simulink model "eml_hdl_design_patterns"  (R2026a)
settings: Solver=FixedStepDiscrete  StopTime=10
InitFcn:
  | errMsg  = ['\n\nThis model is only for demonstration purposes.\n\nPlease do not Simulate or code generate directly from this model. \n\nBefore generating code from this model please do copy the relevant blocks of interest from this model to a new model, place them in a subsystem, build a valid test bench around them.\n\nPlease refer to the example model ''eml_hdl_incrementer'' or HDLCoder documentation'];
  | error(sprintf(errMsg));
undefined symbols (not defined in the file or in its folder): C, gain_val, init_val, lower_limit, maxWordLength, thresh, upper_limit
libraries: simulink x2
(part 3 of 5)

== matlab function eml_hdl_design_patterns/CPU Parts/CPU Controller ==
  settings: sampleTime=1
  settings: fimath=|
      | fimath(...
      | 'RoundMode', 'floor',...
      | 'OverflowMode', 'wrap',...
      | 'ProductMode', 'FullPrecision', 'ProductWordLength', 32,...
      | 'SumMode', 'FullPrecision', 'SumWordLength', 32,...
      | 'CastBeforeSum', true)
  data: data_in input uint8; in_flags input fixdt(0,4,0); master_rst input boolean; shifter_sel output; out_flags output; ALU_func output; print_data output; DM_addr output; DM_r_w output; AC_func output; AC_data output; IR_func output; PC_func output; addr_inc output; IM_read output; hlt output; IR_in input fixdt(0,12,0)
function [shifter_sel, out_flags, ALU_func, ...
    print_data, DM_addr, DM_r_w, AC_func, AC_data, IR_func, ...
    PC_func, addr_inc, IM_read, hlt] = Controller(data_in, in_flags, master_rst, IR_in)
% CPU Controller
%
% The CPU Instruction Set:
% ------------------------
% 
% LDA <loc>: AC = content(<loc>)
% LDAI <loc>: AC = content(content(<loc>))
% AND <loc>: AC = AC & content(<loc>)
% ANDI <loc>: AC = AC & content(content(<loc>))
% ADD <loc>: AC = AC + content(<loc>) + C(flag) 
% ADDI <loc>: AC = AC + content(content(<loc>)) + C(flag)
% SUB <loc>: AC = AC - content(<loc>) - C(flag) 
% SUBI <loc>: AC = AC - content(content(<loc>)) - C(flag)
% JMP <loc>: Jump to <PC + <loc>>
% LI <const>: AC = <const>
% STA <loc>: content(<loc>) = AC
% STAI <loc>: content(content(<loc>)) = AC
% BRA_C <loc>: Jump to <PC + <loc>> if (C(flag) == 1)
% BRA_N <loc>: Jump to <PC + <loc>> if (N(flag) == 1)
% BRA_V <loc>: Jump to <PC + <loc>> if (V(flag) == 1)
% BRA_Z <loc>: Jump to <PC + <loc>> if (Z(flag) == 1)
% NOP: Do nothing
% CLA: AC = 0
% CMA: Complement AC
% CMC: Complement C(flag)
% ASL: AC = AC << 1
% ASR: AC = AC >> 1
% PRINT: Display value from the memory-mapped location 254
% CLC: C(flag) = 0
%
% 12-bit Instruction Encoding:
% ---------------------------
%
% 	LDA:   000 0 <8-bit loc>
% 	LDAI:  000 1 <8-bit loc>
% 	AND:   001 0 <8-bit loc>
% 	ANDI:  001 1 <8-bit loc>
% 	ADD:   010 0 <8-bit loc>
% 	ADDI:  010 1 <8-bit loc>
% 	SUB:   011 0 <8-bit loc>
% 	SUBI:  011 1 <8-bit loc>
% 	JMP:   1000 <8-bit loc>
% 	LI:    1001 <8-bit const>
% 	STA:   101 0 <8-bit loc>
% 	STAI:  101 1 <8-bit loc>
% 	BRA_C: 1100 <8-bit loc>
% 	BRA_N: 1101 <8-bit loc>
% 	BRA_C: 1110 <8-bit loc>
% 	BRA_C: 1111 <8-bit loc>
% 	HLT:   111 0 0100 0 000 
% 	CLA:   111 0 0100 1 000
% 	CMA:   111 0 0101 0 000
% 	CMC:   111 0 0101 1 000
% 	ASL:   111 0 0110 0 000
% 	ASR:   111 0 0110 1 000
% 	PRINT: 111 0 0111 0 000
% 	CLC:   111 0 0111 1 000  

% HDL specific fimath
hdl_fm = fimath(...
'RoundMode', 'floor',...
'OverflowMode', 'wrap',...
'ProductMode', 'FullPrecision', 'ProductWordLength', 32,...
'SumMode', 'FullPrecision', 'SumWordLength', 32,...
'CastBeforeSum', true);


persistent CPU_state;
if(isempty(CPU_state))
    CPU_state = uint8(0);
end

if(master_rst)
    CPU_state = uint8(0);
end

shifter_sel = fi(0, 0, 2, 0, hdl_fm);
ALU_func = fi(0, 0, 3, 0, hdl_fm);
out_flags = in_flags;
AC_func = fi(4, 0, 3, 0, hdl_fm);  % NOP
AC_data = fi(0, 1, 8, 0, hdl_fm);
IR_func = fi(3, 0, 2, 0, hdl_fm);  % NOP
PC_func = fi(3, 0, 2, 0, hdl_fm);  % NOP
IM_read = fi(0, 0, 1, 0, hdl_fm);
DM_addr = uint8(0);
DM_r_w = fi(0, 0, 2, 0, hdl_fm);
addr_inc = fi(0, 1, 8, 0, hdl_fm);
print_data = false;
hlt = uint8(0);

% Instruction: <12..1>
% major_opcode: <12..10>
% indirect_addressing: <9>
% minor_opcode: <9..4>
% address bits: <8..1>

persistent major_opcode; 
persistent minor_opcode; 
persistent address_data;

if(isempty(major_opcode))
    major_opcode = fi(0, 0, 8, 0, hdl_fm);
    minor_opcode = fi(0, 0, 8, 0, hdl_fm);
    address_data = fi(0, 0, 8, 0, hdl_fm);
end

switch(CPU_state)
    %%%%%%%%%%%%%%%%%%%%%%%%%%%%%%%%%%%%%%
    %  RESETTING OUTPUTS
    %%%%%%%%%%%%%%%%%%%%%%%%%%%%%%%%%%%%%%
    case 0
        PC_func = fi(0, 0, 2, 0, hdl_fm);   
        AC_func = fi(0, 0, 3, 0, hdl_fm);   
        IR_func = fi(0, 0, 2, 0, hdl_fm);   
        CPU_state = uint8(1);
        
    %%%%%%%%%%%%%%%%%%%%%%%%%%%%%%%%%%%%%%
    %  FETCH
    %%%%%%%%%%%%%%%%%%%%%%%%%%%%%%%%%%%%%%
    case 1 
        % Read from IM
        IM_read = fi(1, 0, 1, 0, hdl_fm);  
        % Increment PC
        PC_func = fi(2, 0, 2, 0, hdl_fm);  
        % store into IR
        IR_func = fi(1, 0, 2, 0, hdl_fm);  
        CPU_state = uint8(2);
        
    case 2 
        % Read from IR
        IR_func = fi(2, 0, 2, 0, hdl_fm);  
        % Accommodating for the 'unit delay' from IR_out to IR_in
        CPU_state = uint8(3);  
        
    case 3
        % IR_in <12..10>
        major_opcode = fi(bitsrl(IR_in, 9), 0, 8, 0, hdl_fm);
        mask = fi(63, 0, 12, 0, hdl_fm);
        % IR_in <9..4>
        minor_opcode = fi(bitand(bitsrl(IR_in, 3), mask), 0, 8, 0, hdl_fm);
        mask = fi(255, 0, 12, 0, hdl_fm);
        % IR_in <8..1>
        address_data = fi(bitand(IR_in, mask), 0, 8, 0, hdl_fm);
        
        % Go to the decode stage
        CPU_state = uint8(4);  
        
    %%%%%%%%%%%%%%%%%%%%%%%%%%%%%%%%%%%%%%
    %  DECODE AND EXECUTE
    %%%%%%%%%%%%%%%%%%%%%%%%%%%%%%%%%%%%%%
    case 4  
        switch(uint8(major_opcode))
            case 0  
                % LDA
                % minor_opcode contains the address (assuming direct addressing)
                DM_addr = uint8(address_data); 
                % Read the data memory
                DM_r_w = fi(2, 0, 2, 0, hdl_fm); 
                % Simply pass the value read from memory
                ALU_func = fi(6, 0, 3, 0, hdl_fm); 
                shifter_sel = fi(3, 0, 2, 0, hdl_fm); 
                
                indirect_bit = bitget(minor_opcode, 6);
                
                if(logical(indirect_bit))
                    % indirect addressing
                    CPU_state = uint8(7);
                else
                    CPU_state = uint8(6);
                end
                
            case 1  
                % AND           
                DM_addr = uint8(address_data);
                % Reading the data memory for address or data
                DM_r_w = fi(2, 0, 2, 0, hdl_fm);
                indirect_bit = bitget(minor_opcode, 6);
                if(logical(indirect_bit))
                    % indirect addressing
                    CPU_state = uint8(8);
                else
                    % Performing AND
                    ALU_func = fi(1, 0, 3, 0, hdl_fm);
                    shifter_sel = fi(3, 0, 2, 0, hdl_fm);
                    CPU_state = uint8(6);
                end
                
            case 2  
                % ADD
                DM_addr = uint8(address_data);
                % Reading the data memory for address or data
                DM_r_w = fi(2, 0, 2, 0, hdl_fm);
                indirect_bit = bitget(minor_opcode, 6);
                if(logical(indirect_bit))
                    % indirect addressing
                    CPU_state = uint8(9);
                else
                    % Performing ADD
                    ALU_func = fi(2, 0, 3, 0, hdl_fm); 
                    shifter_sel = fi(3, 0, 2, 0, hdl_fm);
                    CPU_state = uint8(6);
                end 
                
            case 3  
                % SUB
                DM_addr = uint8(address_data);
                % Reading the data memory for address or data
                DM_r_w = fi(2, 0, 2, 0, hdl_fm);
                indirect_bit = bitget(minor_opcode, 6);
                if(logical(indirect_bit))
                    % indirect addressing
                    CPU_state = uint8(10);
                else
                    % Performing SUB
                    ALU_func = fi(3, 0, 3, 0, hdl_fm); 
                    shifter_sel = fi(3, 0, 2, 0, hdl_fm);
                    CPU_state = uint8(6);
                end 

            case 4  
                minor_opcode_bit6 = bitget(minor_opcode, 6);
                switch(uint8(minor_opcode_bit6))
                    case 0 
                        % JMP
                        temp_address_data = fi(address_data, 1, 7, 0, hdl_fm);
                        addr_inc = fi(temp_address_data-1, 1, 8, 0, hdl_fm);
                        PC_func = fi(1, 0, 2, 0, hdl_fm); 
                        
                    case 1
                        % LI
                        AC_data = fi(address_data, 1, 8, 0, hdl_fm);
                        AC_func = fi(1, 0, 3, 0, hdl_fm);
                end
                % Go back to the fetch stage again
                CPU_state = uint8(1);  
                
            case 5  
                % STA
                % minor_opcode contains the address (assuming direct addressing)
                DM_addr = uint8(address_data); 
                indirect_bit = bitget(minor_opcode, 6);
                if(logical(indirect_bit))
                    % indirect addressing
                    % Read the address from the data memory
                    DM_r_w = fi(2, 0, 2, 0, hdl_fm); 
                    CPU_state = uint8(11);
                else
                    % Write into the data memory
                    DM_r_w = fi(1, 0, 2, 0, hdl_fm);
                    % Go back to the fetch stage again
                    CPU_state = uint8(1);
                end
                
            case 6
                minor_opcode_bit6 = bitget(minor_opcode, 6);
                switch(uint8(minor_opcode_bit6))
                    % special branches:
                    case 0 
                        % BRA_C
                        c = bitget(in_flags, 4);
                        if(logical(c))
                            temp_address_data = fi(address_data, 1, 7, 0, hdl_fm);
                            addr_inc = fi(temp_address_data-1, 1, 8, 0, hdl_fm);
                            PC_func = fi(1, 0, 2, 0, hdl_fm);
                        end
                        
                    case 1
                        % BRA_N
                        n = bitget(in_flags, 3);
                        if(logical(n))
                            temp_address_data = fi(address_data, 1, 7, 0, hdl_fm);
                            addr_inc = fi(temp_address_data-1, 1, 8, 0, hdl_fm);
                            PC_func = fi(1, 0, 2, 0, hdl_fm);
                        end
                end
                % Go back to the fetch stage again
                CPU_state = uint8(1);
                
            case 7  
                 % by default, go back to the fetch stage again
                CPU_state = uint8(1);
                minor_opcode_bit4 = bitget(minor_opcode, 4);
                if(logical(minor_opcode_bit4) == 0)
                    % Further cases of special branches:
                    minor_opcode_bit6 = bitget(minor_opcode, 6);
                    switch(uint8(minor_opcode_bit6))
                        case 0 
                            % BRA_V
                            v = bitget(in_flags, 2);
                            if(logical(v))
                                temp_address_data = fi(address_data, 1, 7, 0, hdl_fm);
                                addr_inc = fi(temp_address_data-1, 1, 8, 0, hdl_fm);
                                PC_func = fi(1, 0, 2, 0, hdl_fm);
                            end
                         
                        case 1 
                            % BRA_Z
                            z = bitget(in_flags, 1);
                            if(logical(z))
                                temp_address_data = fi(address_data, 1, 7, 0, hdl_fm);
                                addr_inc = fi(temp_address_data-1, 1, 8, 0, hdl_fm);
                                PC_func = fi(1, 0, 2, 0, hdl_fm);
                            end
                    end
                end
                % Instructions having no operands
                switch(uint8(minor_opcode))
                    case 8
                        % HLT
                        % Stop the simulation
                        hlt = uint8(1);
                        CPU_state = uint8(1);
                    case 9 
                        % CLA
                        AC_func = fi(0, 0, 3, 0, hdl_fm);
                        
                    case 10 
                        % CMA
                        ALU_func = fi(4, 0, 3, 0, hdl_fm); 
                        shifter_sel = fi(3, 0, 2, 0, hdl_fm);
                        CPU_state = uint8(6);
                        
                    case 11 
                        % CMC
                        ALU_func = fi(5, 0, 3, 0, hdl_fm); 
                        shifter_sel = fi(3, 0, 2, 0, hdl_fm);
                        
                    case 12 
                        % ASL
                        shifter_sel = fi(1, 0, 2, 0, hdl_fm);
                        CPU_state = uint8(6);
                        
                    case 13 
                        % ASR
                        shifter_sel = fi(2, 0, 2, 0, hdl_fm);
                        CPU_state = uint8(6);
                        
                    case 14 
                        % PRINT
                        print_data = true;
                        
                    case 15 
                        % CLC
                        ALU_func = fi(7, 0, 3, 0, hdl_fm); 
                        shifter_sel = fi(3, 0, 2, 0, hdl_fm);
                        
                    otherwise
                        % by default, go back to the fetch stage again
                        CPU_state = uint8(1);
  
                % Minor Opcode cases end here        
                end
        % Major Opcode cases end here
        end
    
    % introducing delay
    case 6
        % accounting for the delay from shift_out to AC_in2
        AC_func = fi(2, 0, 3, 0, hdl_fm);
        % Go back to the fetch stage again
        CPU_state = uint8(1);  
        
    % Operations with indirect addressing
    case 7
        % LDA Indirect
        % data_in is the address read from the data memory
        DM_addr = uint8(data_in); 
        % Read the data memory
        DM_r_w = fi(2, 0, 2, 0, hdl_fm); 
        % Simply pass the value read from memory
        ALU_func = fi(6, 0, 3, 0, hdl_fm); 
        shifter_sel = fi(3, 0, 2, 0, hdl_fm); 
        % accounting for the algebraic loop delay        
        CPU_state = uint8(6);
        
    case 8
        % AND Indirect
        % data_in is the address read from the data memory
        DM_addr = uint8(data_in);
        % Read the data memory
        DM_r_w = fi(2, 0, 2, 0, hdl_fm);
        % Performing AND
        ALU_func = fi(1, 0, 3, 0, hdl_fm);
        shifter_sel = fi(3, 0, 2, 0, hdl_fm);
        % accounting for the algebraic loop delay
        CPU_state = uint8(6);
    
    case 9
        % ADD Indirect
        % data_in is the address read from the data memory
        DM_addr = uint8(data_in);
        % Read the data memory
        DM_r_w = fi(2, 0, 2, 0, hdl_fm);
        % Performing ADD
        ALU_func = fi(2, 0, 3, 0, hdl_fm); 
        shifter_sel = fi(3, 0, 2, 0, hdl_fm);
        % accounting for the algebraic loop delay
        CPU_state = uint8(6);
        
    case 10
        % SUB Indirect
        % data_in is the address read from the data memory
        DM_addr = uint8(data_in);
        % Read the data memory
        DM_r_w = fi(2, 0, 2, 0, hdl_fm);
        % Performing SUB
        ALU_func = fi(3, 0, 3, 0, hdl_fm); 
        shifter_sel = fi(3, 0, 2, 0, hdl_fm);
        % accounting for the algebraic loop delay
        CPU_state = uint8(6);
        
    case 11
        % STA Indirect
        % data_in is the address read from the data memory
        DM_addr = uint8(data_in);
        % Write the data memory
        DM_r_w = fi(1, 0, 2, 0, hdl_fm);
        CPU_state = uint8(1);
        
    otherwise
        % by default, go back to the fetch stage again
        CPU_state = uint8(1);
                
% switch(CPU_state) end here
end

== matlab function eml_hdl_design_patterns/Misc/const_typing/untyped ==
  settings: fimath=|
      | fimath(...
      | 'RoundMode', 'floor',...
      | 'OverflowMode', 'wrap',...
      | 'ProductMode', 'FullPrecision', 'ProductWordLength', 32,...
      | 'SumMode', 'FullPrecision', 'SumWordLength', 32,...
      | 'CastBeforeSum', true)
  data: u input fixdt(1,14,3); y output
function y = fcn(u)

% based on the internal rule that 
% computes output type gives 
% non-optimial result type (sfix24_En12)

y = u + 1;

== matlab function eml_hdl_design_patterns/Misc/const_typing/typed ==
  settings: fimath=|
      | fimath(...
      | 'RoundMode', 'floor',...
      | 'OverflowMode', 'wrap',...
      | 'ProductMode', 'FullPrecision', 'ProductWordLength', 32,...
      | 'SumMode', 'FullPrecision', 'SumWordLength', 32,...
      | 'CastBeforeSum', true)
  data: u input fixdt(1,14,3); y1 output; y2 output
function [y1, y2] = fcn(u)

% choose minimal required for const 1
y1 = u + fi(1, 0, 1, 0, fimath(u));

% choose same type as var u
y2 = u + fi(1, numerictype(u), fimath(u));

% 
% you get optimal result types (sfix15_En3)
% when you explicitly choose constant types
%
% IMP: Also do not forget to choose 'FullPrecision' 
% on 'Product' and 'SumModes' in the fimath settings
% of this block

== matlab function eml_hdl_design_patterns/Comparators/eml_tree_min ==
  settings: fimath=|
      | fimath(...
      | 'RoundMode', 'floor',...
      | 'OverflowMode', 'wrap',...
      | 'ProductMode', 'FullPrecision', 'ProductWordLength', 32,...
      | 'SumMode', 'FullPrecision', 'SumWordLength', 32,...
      | 'CastBeforeSum', true)
  data: invec input fixdt(1,12,6) size=64; minval output; idx output uint32
%--------------------------------------------------------------------------
% Tree implementation min function for vector input of length 64
%--------------------------------------------------------------------------
function [minval, idx] = fcn(invec)

% initialize outputs
minval = gethdlfi(0, 1, 12, 6);
idx = uint32(0);

% first level of comparison
inidx = uint32(1:64);
[lvlonemin, lvloneidx] = vector_min(invec, inidx);

% second level of comparison
[lvltwomin, lvltwoidx] = vector_min(lvlonemin, lvloneidx);

% third level of comparison
[lvlthreemin, lvlthreeidx] = vector_min(lvltwomin, lvltwoidx);

% fourth level of comparison
[lvlfourmin, lvlfouridx] = vector_min(lvlthreemin, lvlthreeidx);

% fifth level of comparison
[lvlfivemin, lvlfiveidx] = vector_min(lvlfourmin, lvlfouridx);

% final comparison
[minval, idx] = vector_min(lvlfivemin, lvlfiveidx);


end

% Minimum subfuction for tree implementation
function [minvec, idxvec] = vector_min(invec, inidx)
    
lengthminvec = uint8(length(invec)/2);
minvec = gethdlfi(zeros(lengthminvec, 1), 1, 12, 6);
idxvec = uint32(zeros(lengthminvec, 1));

for i=1:lengthminvec
    % get two consecutive values
    idx2 = int8(i)+int8(i); %i*2
    idx1 = int8(idx2) - int8(1); %i*2-1
    % get elements
    val1 = invec(idx1);
    val2 = invec(idx2);
    % compare them and select minimum
    if val1 <= val2
        minvec(i) = val1;
        idxvec(i) = inidx(idx1);
    else
        minvec(i) = val2;
        idxvec(i) = inidx(idx2);
    end
end

end


function myfi = gethdlfi(input, issigned, wlen, flen)

fm = fimath(...
    'RoundMode', 'floor',...
    'OverflowMode', 'wrap',...
    'ProductMode', 'FullPrecision', 'ProductWordLength', 32,...
    'SumMode', 'FullPrecision', 'SumWordLength', 32,...
    'CastBeforeSum', true);

myfi = fi(input, issigned, wlen, flen, 'fimath', fm);

end

== matlab function eml_hdl_design_patterns/Complex/Real Imag To Complex ==
  settings: fimath=|
      | fimath(...
      | 'RoundMode', 'floor',...
      | 'OverflowMode', 'wrap',...
      | 'ProductMode', 'FullPrecision', 'ProductWordLength', 32,...
      | 'SumMode', 'FullPrecision', 'SumWordLength', 32,...
      | 'CastBeforeSum', true)
  data: re input; c output; im input
function c = fcn(re, im)
% Convert real and/or imaginary inputs to complex signal
%
% This Real-Imag to Complex function converts real and/or imaginary inputs
% to a complex-valued output signal.
%
% The inputs can both be arrays (vectors) of equal dimensions, 
% or one input can be an array and the other a scalar. If the function 
% has an array input, the output is a complex array of the 
% same dimensions. 
%
% The elements of the real input are mapped to the real parts of the 
% corresponding complex output elements. The imaginary input is similarly 
% mapped to the imaginary parts of the complex output signals. 
% If one input is a scalar, it is mapped to the corresponding component 
% (real or imaginary) of all the complex output signals. 
%
% The input signals and real or imaginary output parameter can be of any
% data type supported by Simulink, except Boolean. The Real-Imag
% to Complex block supports fixed-point data types. The output is of 
% the same type as the input or parameter that determines the output.

c = complex(re, im);

== matlab function eml_hdl_design_patterns/Misc/eml_expr ==
  settings: fimath=|
      | fimath(...
      | 'RoundMode', 'ceil',...
      | 'OverflowMode', 'saturate',...
      | 'ProductMode', 'FullPrecision', 'ProductWordLength', 32,...
      | 'SumMode', 'FullPrecision', 'SumWordLength', 32,...
      | 'CastBeforeSum', true)
  data: a input fixdt(1,5,2); y output fixdt(1,7,4); b input fixdt(1,5,3)
function y = fcn(a,b)

%------------------------ BLOCK COMMENTS BEGIN ------------------------
%
% The following fixpt expression 
%
%       y = fi((a*b) - (a+b), 1, 7, 4);
%
% with operand and output types 
%
%     a (sfix5_En2), b (sfix5_En3),  y (sfix7_En4) 
%
% and with default fixpt settings on the eML block (ceil,saturate)
%
%  fimath(...
%   'RoundMode', 'ceil',...
%   'OverflowMode', 'saturate',...
%   'ProductMode', 'FullPrecision', 'ProductWordLength', 32,...
%   'SumMode', 'FullPrecision', 'SumWordLength', 32,...
%   'CastBeforeSum', true)
%
% should generate the HDL code based on following intermediate result types
%
%      tmul = a*b (sfix10_En5)
% 
%      t2 = (sfix7_En3) a
%      t3 = (sfix7_En3) b
% 
%      tadd = t2 + t3;
% 
%      t4 = (sfix11_En5) tmul;
%      t5 = (sfix11_En5) tadd;
% 
%      tsub = t4 - t5
% 
%      y = (sfix7_En4) tsub;
% 
%  
%------------------------ BLOCK COMMENTS END ------------------------


% fixpt arithmetic expression
expr = (a*b) - (a+b);

% cast the result to correct output type
y = fi(expr, 1, 7, 4);

== matlab function eml_hdl_design_patterns/CPU Parts/Data Memory (256-Bytes) ==
  settings: sampleTime=1
  settings: fimath=|
      | fimath(...
      | 'RoundMode', 'floor',...
      | 'OverflowMode', 'wrap',...
      | 'ProductMode', 'FullPrecision', 'ProductWordLength', 32,...
      | 'SumMode', 'FullPrecision', 'SumWordLength', 32,...
      | 'CastBeforeSum', true)
  data: indirect input boolean; print_data input boolean; ext_out output; addr input uint8; read_write input fixdt(0,2,0); data_out output fixdt(1,8,0); data_in input fixdt(1,8,0)
function [ext_out, data_out] = fcn(indirect, print_data, addr, read_write, data_in)
% An 8-bit byte-addressable Data Memory
% read_write == 1 => write into DM
% read_write == 2 => read from DM
% print_data == 1 => print data out from memory location 32
% indirect == 1 => Indirect addressing, otherwise direct

% HDL specific fimath
hdl_fm = fimath(...
'RoundMode', 'floor',...
'OverflowMode', 'wrap',...
'ProductMode', 'FullPrecision', 'ProductWordLength', 32,...
'SumMode', 'FullPrecision', 'SumWordLength', 32,...
'CastBeforeSum', true);


persistent data;
if(isempty(data))
    data = fi(zeros(1, 256), 1, 8, 0, hdl_fm);
end

% Data in memory
% data(1) = fi(5, 1, 8, 0, hdl_fm);
% data(2) = fi(6, 1, 8, 0, hdl_fm);

% Get the data for indirect referencing
mem_data = data(addr+1);

% Storing data in memory
if(read_write == 1)
    if(indirect)
        % indirect addressing
        new_addr = uint8(mem_data);
        data(new_addr+1) = data_in;
    else
        % direct addressing
        data(addr+1) = data_in;
    end
end


data_out = fi(0, 1, 8, 0, hdl_fm); 

% Loading from memory
if(read_write == 2)
    if(indirect)
        % indirect addressing
        new_addr = uint8(mem_data);
        data_out = data(new_addr + 1);
    else
        % direct addressing
        data_out = mem_data;
    end
end


ext_out = fi(0, 1, 8, 0, hdl_fm);  

% Printing data out from memory location 256 (memory mapped)
if(print_data)
    ext_out = data(255);
end

== matlab function eml_hdl_design_patterns/Adders/ripple_adder ==
  settings: fimath=|
      | fimath(...
      | 'RoundMode', 'floor',...
      | 'OverflowMode', 'wrap',...
      | 'ProductMode', 'FullPrecision', 'ProductWordLength', 32,...
      | 'SumMode', 'FullPrecision', 'SumWordLength', 32,...
      | 'CastBeforeSum', true)
  data: a input fixdt(0,4,0); s output; b input fixdt(0,4,0); carry output
function [s,carry] = fcn(a,b)

% assuming input is of type ufix4

% An and Bn are typically 1-bit
%(but conceptually can be n-bit numbers)

% each adder adds a delay!

nt = numerictype(0, 1, 0);
fm = fimath(a);

a0 = bitsliceget(a, 1, 1);
a1 = bitsliceget(a, 2, 2);
a2 = bitsliceget(a, 3, 3);
a3 = bitsliceget(a, 4, 4);

b0 = bitsliceget(b, 1, 1);
b1 = bitsliceget(b, 2, 2);
b2 = bitsliceget(b, 3, 3);
b3 = bitsliceget(b, 4, 4);

c_in = fi(0, nt, fm);

% add lsb bits
[s0, c0] = bit_adder(a0, b0, c_in);
% add bits at position '1'
[s1, c1] = bit_adder(a1, b1, c0);
% add bits at position '2'
[s2, c2] = bit_adder(a2, b2, c1);
% add msb bits
[s3, c3] = bit_adder(a3, b3, c2);

% form the final sum
s = bitconcat(bitconcat(bitconcat(s3, s2), s1), s0);

% final carry;
carry = c3;

function [s, c] = bit_adder(abit, bbit, cbit)

r = abit + bbit + cbit;

nt = numerictype(abit);
fm = fimath(abit);

s = fi(bitsliceget(r, 1, 1), nt, fm);
c = fi(bitsliceget(r, 2, 2), nt, fm);

== matlab function eml_hdl_design_patterns/CPU Parts/Arithmetic Logical Unit (8-bit) ==
  settings: sampleTime=1
  settings: fimath=|
      | fimath(...
      | 'RoundMode', 'floor',...
      | 'OverflowMode', 'wrap',...
      | 'ProductMode', 'FullPrecision', 'ProductWordLength', 32,...
      | 'SumMode', 'FullPrecision', 'SumWordLength', 32,...
      | 'CastBeforeSum', true)
  data: in_flags input fixdt(0,4,0); func input fixdt(0,3,0); alu_in input fixdt(1,8,0); AC input fixdt(1,8,0); alu_out output fixdt(1,8,0); out_flags output
function [alu_out, out_flags] = ALU(in_flags, func, alu_in, AC)
% This 8-bit ALU supports the following operations:
% AND (Logical AND), ADD, SUB, CMA (Complement AC), CMC (Complement Carry) and CLC (Clear Carry)
% and appropriately sets a 4-bit flag register, which has the following format:
% [C N V Z]

% HDL specific fimath
hdl_fm = fimath(...
'RoundMode', 'floor',...
'OverflowMode', 'wrap',...
'ProductMode', 'FullPrecision', 'ProductWordLength', 32,...
'SumMode', 'FullPrecision', 'SumWordLength', 32,...
'CastBeforeSum', true);

% Get the carry in
carry = bitsliceget(in_flags, 4, 4); 

% Get the overflow in
overflow = bitsliceget(in_flags, 2, 2);

% Simply pass the AC, when there is no designated func
alu_out = fi(AC, 1, 8, 0, hdl_fm);

% 3-bit encoding of ALU ops, which can potentially support upto 8 operations
% Most of the encodings are unused to comply to Parwan supported ops
switch(uint8(func))
    case 0 % NOP
        % simply pass the AC
    case 1 % AND
        % Bitwise AND
        alu_out = bitand(alu_in, AC);
    case 2 % ADD
        % Add with carry and overflow appropriately set
        [alu_out, carry, overflow] = sum_w_carry(AC, alu_in, carry);
    case 3 % SUB
        % Subtract with borrow (set to carry) and overflow appropriately set
        [alu_out, carry, overflow] = sub_w_borrow(AC, alu_in, carry);
    case 4 % CMA
        % Complement AC
        alu_out = fi(bitcmp(AC), 1, 8, 0, hdl_fm);
    case 5 % CMC
        % Complement Carry
        carry = bitcmp(carry);
    case 6 % Get alu_in out
        % Pass the input
        alu_out = fi(alu_in, 1, 8, 0, hdl_fm);
    case 7 % CLC
        % Clear Carry
        carry = fi(0, 0, 1, 0, hdl_fm); 
end

% Negativity  (N)
sign_bit = getmsb(alu_out); 

% Is Zero? (Z)
is_zero = uint8(~all(alu_out));
zero_ufix1 = fi(is_zero, 0, 1, 0, hdl_fm);

% Set the output flag register [C N V Z]
out_flags = bitconcat(bitconcat(bitconcat(carry, sign_bit), overflow), zero_ufix1);

%%%%%%%%%%%%%%%%%%%%%%%%%%%%%%%%%%%%%%%%%%%%%%%%%%%%%%%%%%%%%%%%


%% Full Subtracter with flag register appropriately set 
% diff = u1 - u2 - b_in = u1 + bitcmp(u2) + bitcmp(b_in)
% appropriately set the borrow and the overflow
function [diff, carry, overflow] = sub_w_borrow(u1, u2, b_in)

[diff, carry, overflow] = sum_w_carry(u1, bitcmp(u2), bitcmp(b_in));
%%%%%%%%%%%%%%%%%%%%%%%%%%%%%%%%%%%%%%%%%%%%%%%%%%%%%%%%%%%%%%%%


%% Full Adder with flag register appropriately set
% sum = u1 + u2 + c_in
% appropriately set the carry and the overflow
function [sum, carry, overflow] = sum_w_carry(u1, u2, c_in)

hdl_fm = fimath(...
'RoundMode', 'floor',...
'OverflowMode', 'wrap',...
'ProductMode', 'FullPrecision', 'ProductWordLength', 32,...
'SumMode', 'FullPrecision', 'SumWordLength', 32,...
'CastBeforeSum', true);

% zero-extend u1 by 1 bit for carry detection
temp_u1 = fi(bitconcat(fi(0, 0, 1, 0, hdl_fm), u1), 1, 9, 0, hdl_fm);

% zero-extend u2 by 1 bit for carry detection
temp_u2 = fi(bitconcat(fi(0, 0, 1, 0, hdl_fm), u2), 1, 9, 0, hdl_fm);

% Sum is stored in 9 bits with the msb indicating carry
temp_sum = fi(temp_u1 + temp_u2 + c_in, 1, 9, 0, hdl_fm);

% Carry  (C)
carry = getmsb(temp_sum);

% Stored back in the designated register
sum = fi(temp_sum, 1, 8, 0, hdl_fm);

% Sign bit
sign_bit = getmsb(sum); 

% if the inputs have the same sign and the output generated has a different sign, 
% overflow is generated!
overflow_int = uint8((getmsb(u1) == getmsb(u2)) ...
                     && (sign_bit ~= bitsliceget(u1,8,8)));
                 
% Overflow (V)
overflow = fi(overflow_int, 0, 1, 0, hdl_fm);

%%%%%%%%%%%%%%%%%%%%%%%%%%%%%%%%%%%%%%%%%%%%%%%%%%%%%%%%%%%%%%%%

== matlab function eml_hdl_design_patterns/Combinatorics/eml_expr ==
  settings: fimath=|
      | fimath(...
      | 'RoundMode', 'ceil',...
      | 'OverflowMode', 'saturate',...
      | 'ProductMode', 'FullPrecision', 'ProductWordLength', 32,...
      | 'SumMode', 'FullPrecision', 'SumWordLength', 32,...
      | 'CastBeforeSum', true)
  data: a input fixdt(1,5,2); y output fixdt(1,7,4); b input fixdt(1,5,3)
function y = fcn(a,b)

%------------------------ BLOCK COMMENTS BEGIN ------------------------
%
% The following fixpt expression 
%
%       y = fi((a*b) - (a+b), 1, 7, 4);
%
% with operand and output types 
%
%     a (sfix5_En2), b (sfix5_En3),  y (sfix7_En4) 
%
% and with default fixpt settings on the eML block (ceil,saturate)
%
%  fimath(...
%   'RoundMode', 'ceil',...
%   'OverflowMode', 'saturate',...
%   'ProductMode', 'FullPrecision', 'ProductWordLength', 32,...
%   'SumMode', 'FullPrecision', 'SumWordLength', 32,...
%   'CastBeforeSum', true)
%
% should generate the HDL code based on following intermediate result types
%
%      tmul = a*b (sfix10_En5)
% 
%      t2 = (sfix7_En3) a
%      t3 = (sfix7_En3) b
% 
%      tadd = t2 + t3;
% 
%      t4 = (sfix11_En5) tmul;
%      t5 = (sfix11_En5) tadd;
% 
%      tsub = t4 - t5
% 
%      y = (sfix7_En4) tsub;
% 
%  
%------------------------ BLOCK COMMENTS END ------------------------


% fixpt arithmetic expression
expr = (a*b) - (a+b);

% cast the result to correct output type
y = fi(expr, 1, 7, 4);

== matlab function eml_hdl_design_patterns/CPU Parts/Shifter (8-bit) ==
  settings: sampleTime=1
  settings: fimath=|
      | fimath(...
      | 'RoundMode', 'floor',...
      | 'OverflowMode', 'wrap',...
      | 'ProductMode', 'FullPrecision', 'ProductWordLength', 32,...
      | 'SumMode', 'FullPrecision', 'SumWordLength', 32,...
      | 'CastBeforeSum', true)
  data: out_flags output; select input fixdt(0,2,0); shift_out output fixdt(1,8,0); input input fixdt(1,8,0); in_flags input fixdt(0,4,0)
function [out_flags, shift_out] = Shifter(select, input, in_flags)
% An 8-bit shifter:
% select = 1 => shift left by 1 bit
% select = 2 => shift right by 1 bit
% otherwise, pass the input

% HDL specific fimath
hdl_fm = fimath(...
'RoundMode', 'floor',...
'OverflowMode', 'wrap',...
'ProductMode', 'FullPrecision', 'ProductWordLength', 32,...
'SumMode', 'FullPrecision', 'SumWordLength', 32,...
'CastBeforeSum', true);

% Overflow (V)
overflow = bitsliceget(in_flags, 2, 2);

% Carry (C)
c_out = bitsliceget(in_flags, 4, 4);

switch(uint8(select))
    case 1
        % shift left
        % affects C and V as well
        shift_out = bitsll(input, 1);
        % Carry (C)
        c_out = bitsliceget(input, 8, 8);
        % Overflow (V)
        overflow = bitxor(bitsliceget(input, 8, 8), bitsliceget(input, 7, 7));
    case 2
        % shift right
        shift_out = bitsra(input, 1);
    otherwise
        % pass the input
        shift_out = fi(input, 1, 8, 0, hdl_fm);
end

% Negativity  (N)
sign_bit = getmsb(shift_out); 

% Is Zero? (Z)
is_zero = uint8(~all(shift_out));
zero_ufix1 = fi(is_zero, 0, 1, 0, hdl_fm);

% Set [C, N, V, Z] in the flag register
out_flags = bitconcat(bitconcat(bitconcat(c_out, sign_bit), overflow), zero_ufix1);

== matlab function eml_hdl_design_patterns/CPU Parts/Accumulator ==
  settings: sampleTime=1
  settings: fimath=|
      | fimath(...
      | 'RoundMode', 'floor',...
      | 'OverflowMode', 'wrap',...
      | 'ProductMode', 'FullPrecision', 'ProductWordLength', 32,...
      | 'SumMode', 'FullPrecision', 'SumWordLength', 32,...
      | 'CastBeforeSum', true)
  data: func input uint8; AC_out output fixdt(1,8,0); AC_in1 input fixdt(1,8,0); AC_in2 input fixdt(1,8,0)

%% Accummulator with the following func:
% func == 0 => reset
% func == 1 => store into AC from port 1
% func == 2 => store into AC from port 2
% func == 3 => read from AC;
% otherwise, preserve old value and return 0
function AC_out = fcn(func, AC_in1, AC_in2)

% HDL specific fimath
hdl_fm = fimath(...
'RoundMode', 'floor',...
'OverflowMode', 'wrap',...
'ProductMode', 'FullPrecision', 'ProductWordLength', 32,...
'SumMode', 'FullPrecision', 'SumWordLength', 32,...
'CastBeforeSum', true);


persistent AC_value;
if(isempty(AC_value))
    AC_value = fi(0, 1, 8, 0, hdl_fm);
end

AC_out = fi(AC_value, 1, 8, 0, hdl_fm);
        
switch(uint8(func)) 
    case 0
        % reset
        AC_value = fi(0, 1, 8, 0, hdl_fm); 
    case 1 
        % store into AC
        AC_value = AC_in1;
    case 2
        % store into AC
        AC_value = AC_in2;    
    case 3
        % read the AC value
        AC_out = AC_value;
end

== matlab function eml_hdl_design_patterns/CPU Parts/Program Counter ==
  settings: sampleTime=1
  settings: fimath=|
      | fimath(...
      | 'RoundMode', 'floor',...
      | 'OverflowMode', 'wrap',...
      | 'ProductMode', 'FullPrecision', 'ProductWordLength', 32,...
      | 'SumMode', 'FullPrecision', 'SumWordLength', 32,...
      | 'CastBeforeSum', true)
  data: func input fixdt(0,2,0); addr_out output; addr_in input fixdt(0,8,0)
function addr_out = fcn(func, addr_in)
% Program Counter
% func = 0 => reset PC
% func = 1 => load PC
% func = 2 => increment PC

% HDL specific fimath
hdl_fm = fimath(...
'RoundMode', 'floor',...
'OverflowMode', 'wrap',...
'ProductMode', 'FullPrecision', 'ProductWordLength', 32,...
'SumMode', 'FullPrecision', 'SumWordLength', 32,...
'CastBeforeSum', true);

persistent PC_value;
if(isempty(PC_value))
    PC_value = fi(0, 0, 8, 0, hdl_fm);
end

addr_out = fi(PC_value, 0, 8, 0, hdl_fm);

switch(uint8(func)) 
    case 0
        % reset
        PC_value = fi(0, 0, 8, 0, hdl_fm); 
    case 1
        % store into PC
        PC_value = addr_in;
    case 2
        % increment PC
        PC_value = fi(PC_value + 1, 0, 8, 0, hdl_fm);
end

== matlab function eml_hdl_design_patterns/CPU Parts/Instruction ROM ==
  settings: sampleTime=1
  settings: fimath=|
      | fimath(...
      | 'RoundMode', 'floor',...
      | 'OverflowMode', 'wrap',...
      | 'ProductMode', 'FullPrecision', 'ProductWordLength', 32,...
      | 'SumMode', 'FullPrecision', 'SumWordLength', 32,...
      | 'CastBeforeSum', true)
  data: addr input uint8; read input fixdt(0,1,0); instr_out output
function instr_out = fcn(addr, read)
%% Instruction Memory

% read == 1 => read from IM

% HDL specific fimath
hdl_fm = fimath(...
'RoundMode', 'floor',...
'OverflowMode', 'wrap',...
'ProductMode', 'FullPrecision', 'ProductWordLength', 32,...
'SumMode', 'FullPrecision', 'SumWordLength', 32,...
'CastBeforeSum', true);


persistent data;
if(isempty(data))
    data = fi(zeros(1, 256), 0, 12, 0, hdl_fm);
end

% ASSEMBLED CODE from sort.in
data(1) = fi(2314, 0, 12, 0, hdl_fm);    % LI 10
data(2) = fi(2560, 0, 12, 0, hdl_fm);    % STA 0
data(3) = fi(2316, 0, 12, 0, hdl_fm);    % LI 12
data(4) = fi(2561, 0, 12, 0, hdl_fm);    % STA 1
data(5) = fi(2322, 0, 12, 0, hdl_fm);    % LI 18
data(6) = fi(2572, 0, 12, 0, hdl_fm);    % STA 12
data(7) = fi(2310, 0, 12, 0, hdl_fm);    % LI 6
data(8) = fi(2573, 0, 12, 0, hdl_fm);    % STA 13
data(9) = fi(2323, 0, 12, 0, hdl_fm);    % LI 19
data(10) = fi(2574, 0, 12, 0, hdl_fm);    % STA 14
data(11) = fi(2555, 0, 12, 0, hdl_fm);    % LI 251
data(12) = fi(2575, 0, 12, 0, hdl_fm);    % STA 15
data(13) = fi(2319, 0, 12, 0, hdl_fm);    % LI 15
data(14) = fi(2576, 0, 12, 0, hdl_fm);    % STA 16
data(15) = fi(2558, 0, 12, 0, hdl_fm);    % LI 254
data(16) = fi(2577, 0, 12, 0, hdl_fm);    % STA 17
data(17) = fi(2306, 0, 12, 0, hdl_fm);    % LI 2
data(18) = fi(2578, 0, 12, 0, hdl_fm);    % STA 18
data(19) = fi(2315, 0, 12, 0, hdl_fm);    % LI 11
data(20) = fi(2579, 0, 12, 0, hdl_fm);    % STA 19
data(21) = fi(2324, 0, 12, 0, hdl_fm);    % LI 20
data(22) = fi(2580, 0, 12, 0, hdl_fm);    % STA 20
data(23) = fi(2314, 0, 12, 0, hdl_fm);    % LI 10
data(24) = fi(2581, 0, 12, 0, hdl_fm);    % STA 21
data(25) = fi(2305, 0, 12, 0, hdl_fm);    % LI 1
data(26) = fi(2562, 0, 12, 0, hdl_fm);    % STA 2
data(27) = fi(2305, 0, 12, 0, hdl_fm);    % LI 1
data(28) = fi(2563, 0, 12, 0, hdl_fm);    % STA 3
data(29) = fi(2305, 0, 12, 0, hdl_fm);    % LI 1
data(30) = fi(2564, 0, 12, 0, hdl_fm);    % STA 4
data(31) = fi(2, 0, 12, 0, hdl_fm);    % LDA 2
data(32) = fi(3704, 0, 12, 0, hdl_fm);    % CLC
data(33) = fi(1540, 0, 12, 0, hdl_fm);    % SUB 4
data(34) = fi(3704, 0, 12, 0, hdl_fm);    % CLC
data(35) = fi(1025, 0, 12, 0, hdl_fm);    % ADD 1
data(36) = fi(2565, 0, 12, 0, hdl_fm);    % STA 5
data(37) = fi(261, 0, 12, 0, hdl_fm);    % LDAI 5
data(38) = fi(2566, 0, 12, 0, hdl_fm);    % STA 6
data(39) = fi(2, 0, 12, 0, hdl_fm);    % LDA 2
data(40) = fi(3704, 0, 12, 0, hdl_fm);    % CLC
data(41) = fi(1025, 0, 12, 0, hdl_fm);    % ADD 1
data(42) = fi(2567, 0, 12, 0, hdl_fm);    % STA 7
data(43) = fi(263, 0, 12, 0, hdl_fm);    % LDAI 7
data(44) = fi(3704, 0, 12, 0, hdl_fm);    % CLC
data(45) = fi(1542, 0, 12, 0, hdl_fm);    % SUB 6
data(46) = fi(3330, 0, 12, 0, hdl_fm);    % BRA_N 2
data(47) = fi(2055, 0, 12, 0, hdl_fm);    % JMP 7
data(48) = fi(2304, 0, 12, 0, hdl_fm);    % LI 0
data(49) = fi(2563, 0, 12, 0, hdl_fm);    % STA 3
data(50) = fi(263, 0, 12, 0, hdl_fm);    % LDAI 7
data(51) = fi(2821, 0, 12, 0, hdl_fm);    % STAI 5
data(52) = fi(6, 0, 12, 0, hdl_fm);    % LDA 6
data(53) = fi(2823, 0, 12, 0, hdl_fm);    % STAI 7
data(54) = fi(2305, 0, 12, 0, hdl_fm);    % LI 1
data(55) = fi(3704, 0, 12, 0, hdl_fm);    % CLC
data(56) = fi(1026, 0, 12, 0, hdl_fm);    % ADD 2
data(57) = fi(2562, 0, 12, 0, hdl_fm);    % STA 2
data(58) = fi(0, 0, 12, 0, hdl_fm);    % LDA 0
data(59) = fi(3704, 0, 12, 0, hdl_fm);    % CLC
data(60) = fi(1538, 0, 12, 0, hdl_fm);    % SUB 2
data(61) = fi(3842, 0, 12, 0, hdl_fm);    % BRA_Z 2
data(62) = fi(2271, 0, 12, 0, hdl_fm);    % JMP -33
data(63) = fi(2305, 0, 12, 0, hdl_fm);    % LI 1
data(64) = fi(2564, 0, 12, 0, hdl_fm);    % STA 4
data(65) = fi(3, 0, 12, 0, hdl_fm);    % LDA 3
data(66) = fi(3704, 0, 12, 0, hdl_fm);    % CLC
data(67) = fi(1540, 0, 12, 0, hdl_fm);    % SUB 4
data(68) = fi(3842, 0, 12, 0, hdl_fm);    % BRA_Z 2
data(69) = fi(2260, 0, 12, 0, hdl_fm);    % JMP -44
data(70) = fi(2304, 0, 12, 0, hdl_fm);    % LI 0
data(71) = fi(2562, 0, 12, 0, hdl_fm);    % STA 2
data(72) = fi(257, 0, 12, 0, hdl_fm);    % LDAI 1
data(73) = fi(2814, 0, 12, 0, hdl_fm);    % STA 254
data(74) = fi(3696, 0, 12, 0, hdl_fm);    % PRINT
data(75) = fi(2305, 0, 12, 0, hdl_fm);    % LI 1
data(76) = fi(3704, 0, 12, 0, hdl_fm);    % CLC
data(77) = fi(1025, 0, 12, 0, hdl_fm);    % ADD 1
data(78) = fi(2561, 0, 12, 0, hdl_fm);    % STA 1
data(79) = fi(2305, 0, 12, 0, hdl_fm);    % LI 1
data(80) = fi(3704, 0, 12, 0, hdl_fm);    % CLC
data(81) = fi(1026, 0, 12, 0, hdl_fm);    % ADD 2
data(82) = fi(2562, 0, 12, 0, hdl_fm);    % STA 2
data(83) = fi(0, 0, 12, 0, hdl_fm);    % LDA 0
data(84) = fi(3704, 0, 12, 0, hdl_fm);    % CLC
data(85) = fi(1538, 0, 12, 0, hdl_fm);    % SUB 2
data(86) = fi(3842, 0, 12, 0, hdl_fm);    % BRA_Z 2
data(87) = fi(2289, 0, 12, 0, hdl_fm);    % JMP -15
data(88) = fi(3648, 0, 12, 0, hdl_fm);    % HLT

% Loading from memory
if(read == 1)
    instr_out = data(addr+1);
else
    instr_out = fi(0, 0, 12, 0, hdl_fm);
end

== matlab function eml_hdl_design_patterns/FFT/fft_blk ==
  settings: fimath=|
      | fimath(...
      | 'RoundMode', 'floor',...
      | 'OverflowMode', 'wrap',...
      | 'ProductMode', 'FullPrecision', 'ProductWordLength', 32,...
      | 'SumMode', 'FullPrecision', 'SumWordLength', 32,...
      | 'CastBeforeSum', true)
  data: u_r input size=32; y output
function y  = fcn(u_r)
% 32point FFT
% Real input and Complex output
% Cooley-Tukey
% Radix-2
% Decimation in Time

% N point FFT involves N/2 stages.
% 


N = 32;

%reverse input order
bu_r = bitrevorder_hdl(u_r);
bu_i = fi(zeros(32, 1), numerictype(u_r), fimath(u_r));

u = complex(bu_r, bu_i);

y = fft32(N, u);

end

%fft32
function x = fft32(N, u)

nt = numerictype(u);
fm = fimath(u);

x = complex(fi(zeros(32,1), nt, fm));

tu1 = fft16(N, u(1:16));
tu2 = fft16(N, u(17:32));

for i=1:16
    tw = twf(N, (i-1));
    twu = hdlfi_mul(tu2(i), tw);
    [x(i), x(i+16)] = bfly2(tu1(i), twu);
end
end

%fft16
function x = fft16(N, u)

nt = numerictype(u);
fm = fimath(u);

x = complex(fi(zeros(16,1), nt, fm));

tu1 = fft8(N, u(1:8));
tu2 = fft8(N, u(9:16));

for i=1:8
    tw = twf(N, (i-1)*2);
    twu = hdlfi_mul(tu2(i) , tw);
    [x(i), x(i+8)] = bfly2(tu1(i), twu);
end
end

%fft8
function x = fft8(N, u)

nt = numerictype(u);
fm = fimath(u);

x = complex(fi(zeros(8,1), nt, fm));

tu1 = fft4(N, u(1:4));
tu2 = fft4(N, u(5:8));

for i=1:4
    tw = twf(N, (i-1)*4);
    twu = hdlfi_mul(tu2(i) , tw);
    [x(i), x(i+4)] = bfly2(tu1(i), twu);
end
end

%fft4
function x = fft4(N, u)

nt = numerictype(u);
fm = fimath(u);

x = complex(fi(zeros(4,1), nt, fm));

tu1 = complex(fi(zeros(2,1), nt, fm));
tu2 = complex(fi(zeros(2,1), nt, fm));

[tu1(1), tu1(2)] = bfly2(u(1), u(2));
[tu2(1), tu2(2)] = bfly2(u(3), u(4));

% typical butterfly structure in an FFT
%
%    u0 --------------> tu0
%               \   /
%                \ /
%                 x
%                / \
%               /   \
%   u1 ---------------> tu1
%        tw         

for i=1:2
    tw = twf(N, (i-1)*8);
    twu = hdlfi_mul(tu2(i) , tw);
    [x(i), x(i+2)] = bfly2(tu1(i), twu);
end
end


function [x, y] = bfly2(u, v)
%% Two element butterfly
% use sum_fm and sum_nt to clamp the result of addition

sum_fm = fimath(...
'RoundMode', 'floor',...
'OverflowMode', 'wrap',...
'ProductMode', 'FullPrecision', 'ProductWordLength', 32,...
'SumMode', 'FullPrecision', 'SumWordLength', 32,...
'CastBeforeSum', true);

sum_nt = numerictype(1, 15, 10);

x = fi(u + v, sum_nt, sum_fm);
y = fi(u - v, sum_nt, sum_fm);

end

function out = hdlfi_mul(in1, in2)
%% Complex fi multiplication
% use mul_fm and mul_nt to clamp the result of multiplication

mul_fm = fimath(...
'RoundMode', 'floor',...
'OverflowMode', 'wrap',...
'ProductMode', 'FullPrecision', 'ProductWordLength', 32,...
'SumMode', 'FullPrecision', 'SumWordLength', 32,...
'CastBeforeSum', true);

mul_nt = numerictype(1,15, 10);

out = fi(in1 * in2, mul_nt, mul_fm);

end

function W = twf(N, k)
%% complex roots of unity (N=32)
%W = exp(-2*pi*1i*k/N)

twf_fm = fimath(...
'RoundMode', 'floor',...
'OverflowMode', 'wrap',...
'ProductMode', 'FullPrecision', 'ProductWordLength', 32,...
'SumMode', 'FullPrecision', 'SumWordLength', 32,...
'CastBeforeSum', true);

twf_nt = numerictype(1,15, 10);


persistent w_N
if isempty(w_N)
    w_N = fi(exp(-2*pi*1i*(0:(N-1))/N).', twf_nt, twf_fm);
end
W = w_N(k+1);

end


function y = bitrevorder_hdl(u) 
% This function reorders elements of 'u' by computing new index positions 
% that have the bit reversed values of the original index position

N = uint32(length(u));

if bitand(N, 1) ~= 0
    error('invalid input, input length must be even');
end

idx_vec = uint32(0:N-1);
len_pow2 = log2(length(u));

fi_idx_vec = fi(idx_vec, 0, len_pow2, 0);

for ii=1:length(fi_idx_vec)  
    fi_idx_vec(ii) = bitreverse(fi_idx_vec(ii));
end

brev_idx = int32(fi_idx_vec)+1;
y = u(brev_idx);

end

function y = bitreverse(u)
t = u;

nt = numerictype(u);
nt2 = floor(nt.WordLength/2);

for ii=1:nt2
    a = bitget(u, ii);
    b = bitget(u, nt.WordLength-ii+1);
    t = bitset(t, ii, b);
    t = bitset(t, nt.WordLength-ii+1, a);
end

y = t;
end

== matlab function eml_hdl_design_patterns/Complex/Complex To Real Imag ==
  settings: fimath=|
      | fimath(...
      | 'RoundMode', 'floor',...
      | 'OverflowMode', 'wrap',...
      | 'ProductMode', 'FullPrecision', 'ProductWordLength', 32,...
      | 'SumMode', 'FullPrecision', 'SumWordLength', 32,...
      | 'CastBeforeSum', true)
  data: re output; c input; im output
function [re, im]= fcn(c)
% Output real and imaginary parts of complex input signal
%
% This Complex to Real-Imag function accepts a complex-valued signal of any
% data type supported by Simulink, including fixed-point data types. It 
% outputs the real and/or imaginary part of the input signal, depending 
% on the setting of the Output parameter. The real outputs are of the 
% same data type as the complex input. 
%
% The input can be an array (vector) of complex signals, 
% in which case the output signals are arrays of the same dimensions. 
% The real array contains the real parts of the corresponding complex 
% input elements. The imaginary output similarly contains the imaginary 
% parts of the input elements.


re = real(c);
im = imag(c);

== matlab function eml_hdl_design_patterns/Misc/discrete_time_integrator ==
  settings: updateMethod=DISCRETE  sampleTime=1
  settings: fimath=|
      | fimath(...
      | 'RoundMode', 'floor',...
      | 'OverflowMode', 'wrap',...
      | 'ProductMode', 'FullPrecision', 'ProductWordLength', 32,...
      | 'SumMode', 'FullPrecision', 'SumWordLength', 32,...
      | 'CastBeforeSum', true)
  data: u input; y output; init_val parameter; gain_val parameter; upper_limit parameter; lower_limit parameter; is_clipped output
function [y, is_clipped] = fcn(u, init_val, gain_val, upper_limit, lower_limit)
% Discrete Time Integrator in MATLAB Function block

%
% Forward Euler method, also known as Forward Rectangular, 
% or left-hand approximation.  The resulting expression for the 
% output of the block at step n is
%
% y(n) = y(n-1) + K * u(n-1)
%


%%%%%%%%%%%
% Setup
%%%%%%%%%%%

% numeric type to clip the accumulator value after each addition
nt = numerictype(u);
fm = fimath(u);

% variable to hold state between consecutive calls to this block
persistent u_state;
if isempty(u_state)
    u_state = fi(init_val, nt, fm);
end

% numeric type to represent -1,1,0 (sfix2)
nt2 = numerictype(1, 2, 0);

% clip flag status
positive_sat_occurred = fi(1, nt2, fm);
negative_sat_occurred = fi(-1, nt2, fm);
no_sat_occurred = fi(0, nt2, fm);

% cast matlab parameters to proper types
gv = fi(gain_val, nt, fm);
ul = fi(upper_limit, nt, fm);
ll = fi(lower_limit, nt, fm);


%%%%%%%%%%%%%%%%%
% Compute Output
%%%%%%%%%%%%%%%%%

if (u_state >= ul)
    t = ul;
    is_clipped = positive_sat_occurred;
elseif (u_state <= ll)
	t = ll;
    is_clipped = negative_sat_occurred;
else    
    t = u_state;
    is_clipped = no_sat_occurred;
end

y = t;


%%%%%%%%%%%%%%%%%
% Update State
%%%%%%%%%%%%%%%%%

tprod = fi(gv * u, nt, fm);
u_state = fi(t + tprod, nt, fm);

== matlab function eml_hdl_design_patterns/Word Twiddlers/Bits2Int ==
  data: u input; y output
function y = fcn(u)
% Converts 1-D array Bits to an Integer

y = bitconcat(u);

== matlab function eml_hdl_design_patterns/Counters/counter_preset_clear ==
  settings: fimath=|
      | fimath(...
      | 'RoundMode', 'floor',...
      | 'OverflowMode', 'saturate',...
      | 'ProductMode', 'FullPrecision', 'ProductWordLength', 32,...
      | 'SumMode', 'FullPrecision', 'SumWordLength', 32,...
      | 'CastBeforeSum', true)
  data: upDown input boolean; clear input boolean; preset input boolean; presetData input fixdt(0,4,0); count output fixdt(0,4,0) size=1
function count  = fcn(upDown, clear, preset, presetData)

% Up/down with synchronous preset and clear.
% With result_fm 'OverflowMode' set to saturate, this counter won't
% roll over.  Set to 'wrap' if rolling over is desirable.

result_nt = numerictype(0,4,0);
result_fm = fimath('OverflowMode', 'saturate', 'RoundMode', 'floor');

persistent count_reg;
if isempty(count_reg)
    count_reg = fi(0, result_nt, result_fm);
end

count = count_reg;

if clear
    count_reg = fi(0, result_nt, result_fm);
elseif preset
    count_reg = presetData;
elseif upDown
    inc = count_reg + fi(1, result_nt, result_fm);
    count_reg = fi(inc, result_nt, result_fm);
else
    dec = count_reg - fi(1, result_nt, result_fm);
    count_reg = fi(dec, result_nt, result_fm);
end

== matlab function eml_hdl_design_patterns/Decoders/hierarchical_viterbi/BMU1 ==
  settings: fimath=|
      | fimath(...
      | 'RoundMode', 'floor',...
      | 'OverflowMode', 'wrap',...
      | 'ProductMode', 'FullPrecision', 'ProductWordLength', 32,...
      | 'SumMode', 'FullPrecision', 'SumWordLength', 32,...
      | 'CastBeforeSum', true)
  data: u input fixdt(1,6,3) size=2; bm output
function bm = BMU(u)
%--------------------------------------------------------------------------
% Viterbi Decoder Demo
% 
% This model implements viterbi decoder with MATLAB Function blocks.
% The Viterbi Decoder block decodes fixed-point input symbols to produce 
% binary output symbols.
%--------------------------------------------------------------------------

% input symbol
u1 = u(1);
u2 = u(2);

%--------------------------------------------------------------------------
% BMC (Branch Metric) Unit
% This block calculates the Branch Metric (Hamming distance) of input symbols.
% The input are the quantized fixed-point symbols in the form of sfix6_En3.
%--------------------------------------------------------------------------
bm = getfi_sat(zeros(1,4), 1, 12, 6);

%----------------------------
% Hamming distace for (1,1)
%----------------------------
bm(1) = (u1-1)*(u1-1) + (u2-1)*(u2-1);

%----------------------------
% Hamming distace for (1,-1)
%----------------------------
bm(2) = (u1-1)*(u1-1) + (u2-(-1))*(u2-(-1));

%----------------------------
% Hamming distace for (-1,1)
%----------------------------
bm(3) = (u1-(-1))*(u1-(-1)) + (u2-1)*(u2-1);

%----------------------------
% Hamming distace for (-1,-1)
%----------------------------
bm(4) = (u1-(-1))*(u1-(-1)) + (u2-(-1))*(u2-(-1));

end

function myfi = getfi_sat(input, issigned, wlen, flen)

fm_sat = fimath(...
    'RoundMode', 'floor',...
    'OverflowMode', 'saturate',...
    'ProductMode', 'FullPrecision', 'ProductWordLength', 32,...
    'SumMode', 'FullPrecision', 'SumWordLength', 32,...
    'CastBeforeSum', true);

myfi = fi(input, issigned, wlen, flen, 'fimath', fm_sat);

end

== matlab function eml_hdl_design_patterns/Filters/sfir_pipelined ==
  settings: fimath=|
      | fimath(...
      | 'RoundMode', 'floor',...
      | 'OverflowMode', 'wrap',...
      | 'ProductMode', 'FullPrecision',...
      | 'SumMode', 'FullPrecision',...
      | 'CastBeforeSum', true)
  data: x_in input fixdt(1,6,3); y_out output; h_in1 input fixdt(1,6,3); h_in2 input fixdt(1,6,3); h_in3 input fixdt(1,6,3); h_in4 input fixdt(1,6,3)
function y_out  = fcn(x_in, h_in1, h_in2, h_in3, h_in4)
% This block supports an embeddable subset of the MATLAB language.
% See the help menu for details. 

persistent delay;
persistent pipeline;

if isempty(delay)
    delay = fi(zeros(1,8), numerictype(x_in), fimath(x_in));
end

if isempty(pipeline)
    pipeline = fi(zeros(1,4), numerictype(x_in), fimath(x_in));
end

add1 = delay(1) + delay(8);
add2 = delay(2) + delay(7);
add3 = delay(3) + delay(6);
add4 = delay(4) + delay(5);

prod1 = add1 * h_in1;
prod2 = add2 * h_in2;
prod3 = add3 * h_in3;
prod4 = add4 * h_in4;

add5 = pipeline(1) + pipeline(2);
add6 = pipeline(3) + pipeline(4);
add7 = add5 + add6;

y_out = add7;

delay = [x_in delay(1:7)];
pipeline(:) = [prod1 prod2 prod3 prod4];

== matlab function eml_hdl_design_patterns/Complex/Complex Conjugate ==
  settings: fimath=|
      | fimath(...
      | 'RoundMode', 'floor',...
      | 'OverflowMode', 'wrap',...
      | 'ProductMode', 'FullPrecision', 'ProductWordLength', 32,...
      | 'SumMode', 'FullPrecision', 'SumWordLength', 32,...
      | 'CastBeforeSum', true)
  data: cc output; c input
function cc = fcn(c)
% Compute Complex conjugate of c
% For a complex c, conj(c) = real(c) - i * imag(c).

cc = conj(c);

== matlab function eml_hdl_design_patterns/Comparators/eml_linear_min ==
  settings: fimath=|
      | fimath(...
      | 'RoundMode', 'floor',...
      | 'OverflowMode', 'wrap',...
      | 'ProductMode', 'FullPrecision', 'ProductWordLength', 32,...
      | 'SumMode', 'FullPrecision', 'SumWordLength', 32,...
      | 'CastBeforeSum', true)
  data: invec input fixdt(1,12,6) size=8; minval output; idx output
function [minval, idx] = fcn(invec)

% assuming vector length to be 8
% the following calls implement a linear comparison

% level 1
[t1, idx1] = hdl_min(invec(1), invec(2), uint8(1), uint8(2));
% level 2
[t2, idx2] = hdl_min(t1, invec(3), idx1, uint8(3));
% level 3
[t3, idx3] = hdl_min(t2, invec(4), idx2, uint8(4));
% level 4
[t4, idx4] = hdl_min(t3, invec(5), idx3, uint8(5));
% level 5
[t5, idx5] = hdl_min(t4, invec(6), idx4, uint8(6));
% level 6
[t6, idx6] = hdl_min(t5, invec(7), idx5, uint8(7));
% level 7
[minval, idx] = hdl_min(t6, invec(8), idx6, uint8(8));

end

% Minimum subfuction for tree implementation
function [minvec, idxvec] = hdl_min(in1, in2, idx1, idx2)
    
    % compare them and select minimum
    if in1 < in2
        minvec = in1;
        idxvec = idx1;
    else
        minvec = in2;
        idxvec = idx2;
    end
end

function myfi = gethdlfi(input, issigned, wlen, flen)

fm = fimath(...
    'RoundMode', 'floor',...
    'OverflowMode', 'wrap',...
    'ProductMode', 'FullPrecision', 'ProductWordLength', 32,...
    'SumMode', 'FullPrecision', 'SumWordLength', 32,...
    'CastBeforeSum', true);

myfi = fi(input, issigned, wlen, flen, 'fimath', fm);

end
